simulink model "acc_plant"  (R2026b)
settings: Solver=ode3  StopTime=60  FixedStep=0.005
values from neighbouring files (symbols this model uses):
  P = min(P / (lam + pk^2 * P), P0)    [acc_mass_estimate.m]    (also in acc_plant_params.m = longitudinal_params("trailer"); acc_scenario_input.m = acc_plant_params(); build_acc_closed_loop.m = acc_plant_params(); build_acc_plant.m = acc_plant_params())
libraries: simulink x11, sl_discontinuities x2
settings Model: Creator=kikiw  LastModifiedBy=kikiw
settings DebuggingCC: AlgebraicLoopMsg=error

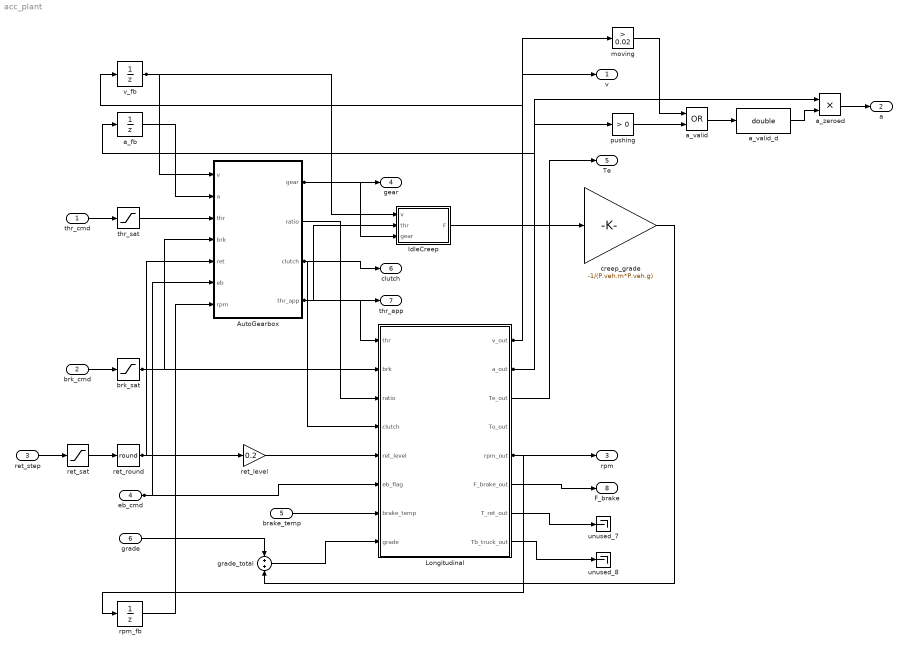
== system acc_plant ==
  thr_cmd : Inport
  brk_cmd : Inport  Port=2
  ret_step : Inport  Port=3
  eb_cmd : Inport  Port=4
  brake_temp : Inport  Port=5
  grade : Inport  Port=6
  AutoGearbox : Stateflow chart  TreatAsAtomicUnit=on
  IdleCreep : MATLAB Function  TreatAsAtomicUnit=on
  Longitudinal : Subsystem
  a_fb : UnitDelay  InitialCondition=P.init.a0  SampleTime=0.02
  a_valid : Logic  Operator=OR  AllPortsSameDT=off  OutDataTypeStr=boolean
  a_valid_d : DataTypeConversion  OutDataTypeStr=double  SaturateOnIntegerOverflow=off  RndMeth=Floor
  a_zeroed : Product
  brk_sat : Saturate  UpperLimit=1  LowerLimit=0
  creep_grade : Gain  Gain=-1/(P.veh.m*P.veh.g)
  grade_total : Sum
  moving : simulink/Logic and Bit Operations/Compare To Constant  relop=>  const=0.02  OutDataTypeStr=boolean
  pushing : simulink/Logic and Bit Operations/Compare To Constant  relop=>  const=0  OutDataTypeStr=boolean
  ret_level : Gain  Gain=0.2
  ret_round : Rounding  Operator=round
  ret_sat : Saturate  UpperLimit=5  LowerLimit=0
  rpm_fb : UnitDelay  InitialCondition=P.init.we0*30/pi  SampleTime=0.02
  thr_sat : Saturate  UpperLimit=1  LowerLimit=0
  unused_7 : Terminator
  unused_8 : Terminator
  v_fb : UnitDelay  InitialCondition=P.init.v0  SampleTime=0.02
  v : Outport
  a : Outport  Port=2
  rpm : Outport  Port=3
  gear : Outport  Port=4
  Te : Outport  Port=5
  clutch : Outport  Port=6
  thr_app : Outport  Port=7
  F_brake : Outport  Port=8
  wires:
  brk_cmd/1 -> brk_sat/1
  moving/1 -> a_valid/1
  ret_step/1 -> ret_sat/1
  AutoGearbox/2(ratio) -> Longitudinal/3(ratio)
  thr_cmd/1 -> thr_sat/1
  ret_sat/1 -> ret_round/1
  a_fb/1 -> AutoGearbox/2(a)
  v_fb/1 -> IdleCreep/1(v), AutoGearbox/1(v)
  thr_sat/1 -> AutoGearbox/3(thr)
  brk_sat/1 -> Longitudinal/2(brk), AutoGearbox/4(brk)
  ret_round/1 -> ret_level/1, AutoGearbox/5(ret)
  eb_cmd/1 -> Longitudinal/6(eb_flag), AutoGearbox/6(eb)
  Longitudinal/1(v_out) -> moving/1, v_fb/1, v/1
  grade/1 -> grade_total/1
  rpm_fb/1 -> AutoGearbox/7(rpm)
  AutoGearbox/1(gear) -> IdleCreep/3(gear), gear/1
  AutoGearbox/3(clutch) -> Longitudinal/4(clutch), clutch/1
  AutoGearbox/4(thr_app) -> Longitudinal/1(thr), IdleCreep/2(thr), thr_app/1
  a_valid_d/1 -> a_zeroed/2
  Longitudinal/8(Tb_truck_out) -> unused_8/1
  ret_level/1 -> Longitudinal/5(ret_level)
  brake_temp/1 -> Longitudinal/7(brake_temp)
  IdleCreep/1(F) -> creep_grade/1
  grade_total/1 -> Longitudinal/8(grade)
  Longitudinal/2(a_out) -> a_fb/1, a_zeroed/1, pushing/1
  Longitudinal/3(Te_out) -> Te/1
  Longitudinal/5(rpm_out) -> rpm_fb/1, rpm/1
  Longitudinal/6(F_brake_out) -> F_brake/1
  Longitudinal/7(T_ret_out) -> unused_7/1
  pushing/1 -> a_valid/2
  creep_grade/1 -> grade_total/2
  a_valid/1 -> a_valid_d/1
  a_zeroed/1 -> a/1

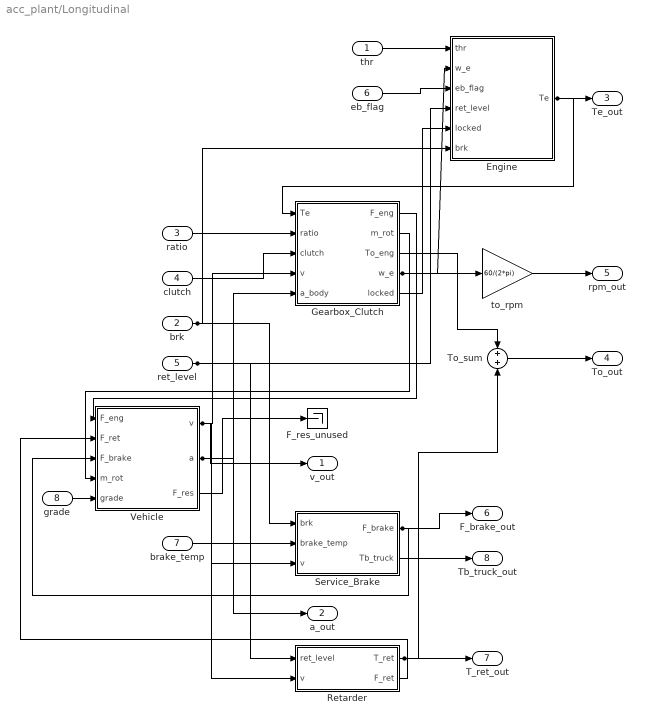
== system acc_plant/Longitudinal ==
  thr : Inport
  brk : Inport  Port=2
  ratio : Inport  Port=3
  clutch : Inport  Port=4
  ret_level : Inport  Port=5
  eb_flag : Inport  Port=6
  brake_temp : Inport  Port=7
  grade : Inport  Port=8
  Engine : Subsystem
  F_res_unused : Terminator
  Gearbox_Clutch : Subsystem
  Retarder : Subsystem
  Service_Brake : Subsystem
  To_sum : Sum
  Vehicle : Subsystem
  to_rpm : Gain  Gain=60/(2*pi)
  v_out : Outport
  a_out : Outport  Port=2
  Te_out : Outport  Port=3
  To_out : Outport  Port=4
  rpm_out : Outport  Port=5
  F_brake_out : Outport  Port=6
  T_ret_out : Outport  Port=7
  Tb_truck_out : Outport  Port=8
  wires:
  grade/1 -> Vehicle/5(grade)
  ratio/1 -> Gearbox_Clutch/2(ratio)
  clutch/1 -> Gearbox_Clutch/3(clutch)
  brk/1 -> Service_Brake/1(brk), Engine/6(brk)
  ret_level/1 -> Retarder/1(ret_level), Engine/4(ret_level)
  Vehicle/3(F_res) -> F_res_unused/1
  Vehicle/1(v) -> Gearbox_Clutch/4(v), Service_Brake/3(v), v_out/1, Retarder/2(v)
  Vehicle/2(a) -> a_out/1, Gearbox_Clutch/5(a_body)
  brake_temp/1 -> Service_Brake/2(brake_temp)
  Gearbox_Clutch/3(To_eng) -> To_sum/1
  thr/1 -> Engine/1(thr)
  eb_flag/1 -> Engine/3(eb_flag)
  Gearbox_Clutch/1(F_eng) -> Vehicle/1(F_eng)
  Gearbox_Clutch/2(m_rot) -> Vehicle/4(m_rot)
  Gearbox_Clutch/4(w_e) -> to_rpm/1, Engine/2(w_e)
  To_sum/1 -> To_out/1
  Gearbox_Clutch/5(locked) -> Engine/5(locked)
  Service_Brake/1(F_brake) -> F_brake_out/1, Vehicle/3(F_brake)
  Service_Brake/2(Tb_truck) -> Tb_truck_out/1
  Retarder/1(T_ret) -> T_ret_out/1, To_sum/2
  Retarder/2(F_ret) -> Vehicle/2(F_ret)
  Engine/1(Te) -> Te_out/1, Gearbox_Clutch/1(Te)
  to_rpm/1 -> rpm_out/1

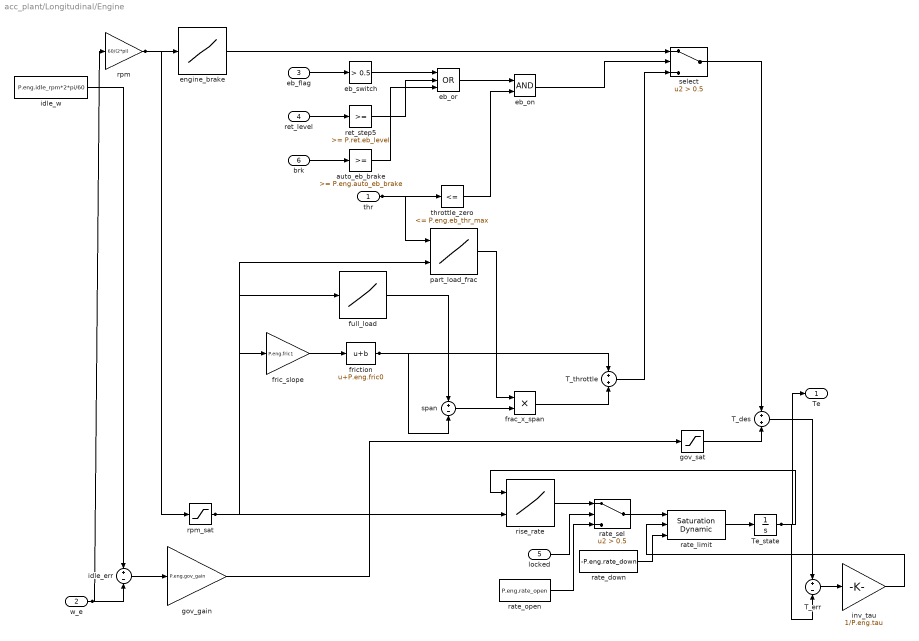
== system acc_plant/Longitudinal/Engine ==
  thr : Inport
  w_e : Inport  Port=2
  eb_flag : Inport  Port=3
  ret_level : Inport  Port=4
  locked : Inport  Port=5
  brk : Inport  Port=6
  T_des : Sum
  T_err : Sum  Inputs=+-
  T_throttle : Sum
  Te_state : Integrator  InitialCondition=P.init.Te0
  auto_eb_brake : simulink/Logic and Bit Operations/Compare To Constant  relop=>=  const=P.eng.auto_eb_brake  OutDataTypeStr=boolean
  eb_on : Logic  AllPortsSameDT=off  OutDataTypeStr=boolean
  eb_or : Logic  Operator=OR  Inputs=3  AllPortsSameDT=off  OutDataTypeStr=boolean
  eb_switch : simulink/Logic and Bit Operations/Compare To Constant  relop=>  const=0.5  OutDataTypeStr=boolean
  engine_brake : Lookup_n-D  NumberOfTableDimensions=1  BreakpointsForDimension1=P.eng.eb_rpm  Table=P.eng.eb_nm  ExtrapMethod=Clip  InternalRulePriority=Speed  RndMeth=Simplest
  frac_x_span : Product
  fric_slope : Gain  Gain=P.eng.fric1
  friction : Bias  Bias=P.eng.fric0  SaturateOnIntegerOverflow=off
  full_load : Lookup_n-D  NumberOfTableDimensions=1  BreakpointsForDimension1=P.eng.curve_rpm  Table=P.eng.T_max*P.eng.curve_frac  ExtrapMethod=Clip  InternalRulePriority=Speed  RndMeth=Simplest
  gov_gain : Gain  Gain=P.eng.gov_gain
  gov_sat : Saturate  UpperLimit=P.eng.T_max  LowerLimit=0
  idle_err : Sum  Inputs=+-
  idle_w : Constant  Value=P.eng.idle_rpm*2*pi/60
  inv_tau : Gain  Gain=1/P.eng.tau
  part_load_frac : Lookup_n-D  BreakpointsForDimension1=P.eng.thr_bp  BreakpointsForDimension2=P.eng.rpm_bp  Table=P.eng.frac_table  ExtrapMethod=Clip  InternalRulePriority=Speed  RndMeth=Simplest
      settings: InputPortMap=u0,u1
  rate_down : Constant  Value=-P.eng.rate_down
  rate_limit : sl_discontinuities/Saturation Dynamic  OutMin=[]  OutMax=[]  OutDataTypeStr=Inherit: Same as second input  OutDataType=fixdt(1, 16)  OutScaling=2^-10  DoSatur=off
      settings: LibrarySourceBlock=|
      | simulink/Discontinuities/Saturation
      | Dynamic
  rate_open : Constant  Value=P.eng.rate_open
  rate_sel : Switch  Criteria=u2 > Threshold  Threshold=0.5  SaturateOnIntegerOverflow=off  InputSameDT=off
  ret_step5 : simulink/Logic and Bit Operations/Compare To Constant  relop=>=  const=P.ret.eb_level  OutDataTypeStr=boolean
  rise_rate : Lookup_n-D  BreakpointsForDimension1=P.eng.rate_te_bp  BreakpointsForDimension2=P.eng.rate_rpm_bp  Table=P.eng.rate_up_table  ExtrapMethod=Clip  InternalRulePriority=Speed  RndMeth=Simplest
      settings: InputPortMap=u0,u1
  rpm : Gain  Gain=60/(2*pi)
  rpm_sat : Saturate  UpperLimit=P.eng.curve_rpm(end)  LowerLimit=P.eng.curve_rpm(1)
  select : Switch  Criteria=u2 > Threshold  Threshold=0.5  SaturateOnIntegerOverflow=off  InputSameDT=off
  span : Sum  Inputs=+-
  throttle_zero : simulink/Logic and Bit Operations/Compare To Constant  relop=<=  const=P.eng.eb_thr_max  OutDataTypeStr=boolean
  Te : Outport
  wires:
  inv_tau/1 -> rate_limit/2
  T_des/1 -> T_err/1
  gov_sat/1 -> T_des/2
  rate_down/1 -> rate_limit/3
  T_err/1 -> inv_tau/1
  rate_sel/1 -> rate_limit/1
  rate_open/1 -> rate_sel/3
  locked/1 -> rate_sel/2
  frac_x_span/1 -> T_throttle/2
  T_throttle/1 -> select/3
  eb_on/1 -> select/2
  rate_limit/1 -> Te_state/1
  span/1 -> frac_x_span/2
  friction/1 -> span/2, T_throttle/1
  part_load_frac/1 -> frac_x_span/1
  full_load/1 -> span/1
  thr/1 -> throttle_zero/1, part_load_frac/1
  rise_rate/1 -> rate_sel/1
  auto_eb_brake/1 -> eb_or/3
  throttle_zero/1 -> eb_on/2
  eb_switch/1 -> eb_or/1
  ret_step5/1 -> eb_or/2
  fric_slope/1 -> friction/1
  eb_or/1 -> eb_on/1
  brk/1 -> auto_eb_brake/1
  ret_level/1 -> ret_step5/1
  eb_flag/1 -> eb_switch/1
  engine_brake/1 -> select/1
  rpm/1 -> engine_brake/1, rpm_sat/1
  rpm_sat/1 -> rise_rate/2, fric_slope/1, full_load/1, part_load_frac/2
  idle_w/1 -> idle_err/1
  Te_state/1 -> T_err/2, Te/1, rise_rate/1
  idle_err/1 -> gov_gain/1
  w_e/1 -> rpm/1, idle_err/2
  select/1 -> T_des/1
  gov_gain/1 -> gov_sat/1

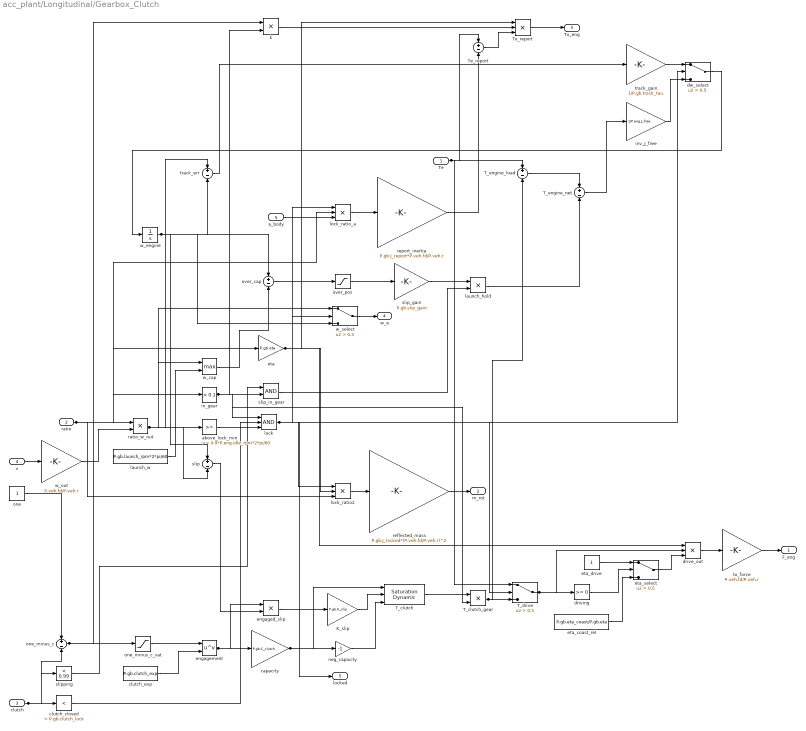
== system acc_plant/Longitudinal/Gearbox_Clutch ==
  Te : Inport
  ratio : Inport  Port=2
  clutch : Inport  Port=3
  v : Inport  Port=4
  a_body : Inport  Port=5
  K_slip : Gain  Gain=P.gb.K_slip
  T_clutch : sl_discontinuities/Saturation Dynamic  OutMin=[]  OutMax=[]  OutDataTypeStr=Inherit: Same as second input  OutDataType=fixdt(1, 16)  OutScaling=2^-10  DoSatur=off
      settings: LibrarySourceBlock=|
      | simulink/Discontinuities/Saturation
      | Dynamic
  T_clutch_gear : Product
  T_drive : Switch  Criteria=u2 > Threshold  Threshold=0.5  SaturateOnIntegerOverflow=off  InputSameDT=off
  T_engine_load : Sum  Inputs=+-
  T_engine_net : Sum  Inputs=+-
  Te_report : Sum  Inputs=+-
  To_report : Product  Inputs=3
  above_lock_min : simulink/Logic and Bit Operations/Compare To Constant  relop=>=  const=0.9*P.eng.idle_rpm*2*pi/60  OutDataTypeStr=boolean
  capacity : Gain  Gain=P.gb.C_clutch
  clutch_closed : simulink/Logic and Bit Operations/Compare To Constant  relop=<  const=P.gb.clutch_lock  OutDataTypeStr=boolean
  clutch_exp : Constant  Value=P.gb.clutch_exp
  drive_out : Product  Inputs=3
  driving : simulink/Logic and Bit Operations/Compare To Constant  relop=>=  const=0  OutDataTypeStr=boolean
  dw_select : Switch  Criteria=u2 > Threshold  Threshold=0.5  SaturateOnIntegerOverflow=off  InputSameDT=off
  engaged_slip : Product
  engagement : Math  Operator=pow
  eta : Gain  Gain=P.gb.eta
  eta_coast_rel : Constant  Value=P.gb.eta_coast/P.gb.eta
  eta_drive : Constant
  eta_select : Switch  Criteria=u2 > Threshold  Threshold=0.5  SaturateOnIntegerOverflow=off  InputSameDT=off
  in_gear : simulink/Logic and Bit Operations/Compare To Constant  relop=>  const=0.1  OutDataTypeStr=boolean
  inv_J_free : Gain  Gain=1/P.eng.J_free
  k : Product
  launch_hold : Product
  launch_w : Constant  Value=P.gb.launch_rpm*2*pi/60
  lock : Logic  Inputs=3  AllPortsSameDT=off  OutDataTypeStr=boolean
  lock_ratio2 : Product  Inputs=3
  lock_ratio_a : Product  Inputs=3
  neg_capacity : Gain  Gain=-1
  one : Constant
  one_minus_c : Sum  Inputs=+-
  one_minus_c_sat : Saturate  UpperLimit=1  LowerLimit=0
  over_cap : Sum  Inputs=+-
  over_pos : Saturate  UpperLimit=inf  LowerLimit=0
  ratio_w_out : Product
  reflected_mass : Gain  Gain=P.gb.J_locked*(P.veh.fd/P.veh.r)^2
  report_inertia : Gain  Gain=P.gb.J_report*P.veh.fd/P.veh.r
  slip : Sum  Inputs=+-
  slip_gain : Gain  Gain=P.gb.slip_gain
  slip_in_gear : Logic  AllPortsSameDT=off  OutDataTypeStr=boolean
  slipping : simulink/Logic and Bit Operations/Compare To Constant  relop=<  const=0.99  OutDataTypeStr=boolean
  to_force : Gain  Gain=P.veh.fd/P.veh.r
  track_err : Sum  Inputs=+-
  track_gain : Gain  Gain=1/P.gb.track_tau
  w_cap : MinMax  Function=max  Inputs=2
  w_engine : Integrator  InitialCondition=P.init.we0  LimitOutput=on  UpperSaturationLimit=P.eng.max_rpm*2*pi/60  LowerSaturationLimit=0
  w_out : Gain  Gain=P.veh.fd/P.veh.r
  w_select : Switch  Criteria=u2 > Threshold  Threshold=0.5  SaturateOnIntegerOverflow=off  InputSameDT=off
  F_eng : Outport
  m_rot : Outport  Port=2
  To_eng : Outport  Port=3
  w_e : Outport  Port=4
  locked : Outport  Port=5
  wires:
  drive_out/1 -> to_force/1
  dw_select/1 -> w_engine/1
  eta_select/1 -> drive_out/3
  inv_J_free/1 -> dw_select/3
  track_gain/1 -> dw_select/1
  eta_coast_rel/1 -> eta_select/3
  driving/1 -> eta_select/2
  eta_drive/1 -> eta_select/1
  T_engine_net/1 -> inv_J_free/1
  T_drive/1 -> driving/1, drive_out/2
  launch_hold/1 -> T_engine_net/2
  T_clutch/1 -> T_clutch_gear/1
  report_inertia/1 -> Te_report/2
  to_force/1 -> F_eng/1
  K_slip/1 -> T_clutch/2
  lock_ratio2/1 -> reflected_mass/1
  slip_gain/1 -> launch_hold/1
  Te_report/1 -> To_report/3
  over_pos/1 -> slip_gain/1
  lock_ratio_a/1 -> report_inertia/1
  To_report/1 -> To_eng/1
  slip_in_gear/1 -> launch_hold/2
  eta/1 -> lock_ratio2/2, To_report/1, drive_out/1
  T_clutch_gear/1 -> T_drive/3, T_engine_load/2
  over_cap/1 -> over_pos/1
  a_body/1 -> lock_ratio_a/3
  k/1 -> To_report/2
  reflected_mass/1 -> m_rot/1
  engagement/1 -> capacity/1, engaged_slip/1
  slip/1 -> engaged_slip/2
  Te/1 -> T_engine_load/1, T_drive/1, Te_report/1
  above_lock_min/1 -> lock/3
  w_cap/1 -> over_cap/2
  in_gear/1 -> k/2, slip_in_gear/2, T_clutch_gear/2, lock/1
  T_engine_load/1 -> T_engine_net/1
  track_err/1 -> track_gain/1
  lock/1 -> locked/1, T_drive/2, lock_ratio2/1, w_select/2, lock_ratio_a/1, dw_select/2
  w_select/1 -> w_e/1
  clutch_exp/1 -> engagement/2
  neg_capacity/1 -> T_clutch/3
  one_minus_c_sat/1 -> engagement/1
  launch_w/1 -> w_cap/2
  ratio_w_out/1 -> w_cap/1, above_lock_min/1, slip/2, w_select/1, track_err/1
  w_engine/1 -> slip/1, over_cap/1, w_select/3, track_err/2
  clutch_closed/1 -> lock/2
  w_out/1 -> ratio_w_out/2
  one/1 -> one_minus_c/1
  one_minus_c/1 -> one_minus_c_sat/1, k/1
  slipping/1 -> slip_in_gear/1
  v/1 -> w_out/1
  capacity/1 -> neg_capacity/1, T_clutch/1
  clutch/1 -> slipping/1, one_minus_c/2, clutch_closed/1
  engaged_slip/1 -> K_slip/1
  ratio/1 -> ratio_w_out/1, lock_ratio_a/2, lock_ratio2/3, eta/1, in_gear/1

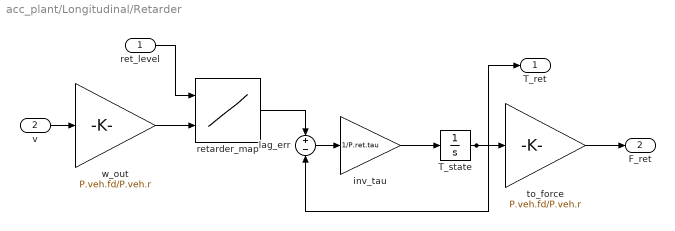
== system acc_plant/Longitudinal/Retarder ==
  ret_level : Inport
  v : Inport  Port=2
  T_state : Integrator  InitialCondition=P.init.ret0
  inv_tau : Gain  Gain=1/P.ret.tau
  lag_err : Sum  Inputs=+-
  retarder_map : Lookup_n-D  BreakpointsForDimension1=P.ret.level_bp  BreakpointsForDimension2=P.ret.w_bp  Table=P.ret.table  ExtrapMethod=Clip  InternalRulePriority=Speed  RndMeth=Simplest
      settings: InputPortMap=u0,u1
  to_force : Gain  Gain=P.veh.fd/P.veh.r
  w_out : Gain  Gain=P.veh.fd/P.veh.r
  T_ret : Outport
  F_ret : Outport  Port=2
  wires:
  ret_level/1 -> retarder_map/1
  inv_tau/1 -> T_state/1
  to_force/1 -> F_ret/1
  v/1 -> w_out/1
  w_out/1 -> retarder_map/2
  retarder_map/1 -> lag_err/1
  lag_err/1 -> inv_tau/1
  T_state/1 -> to_force/1, T_ret/1, lag_err/2

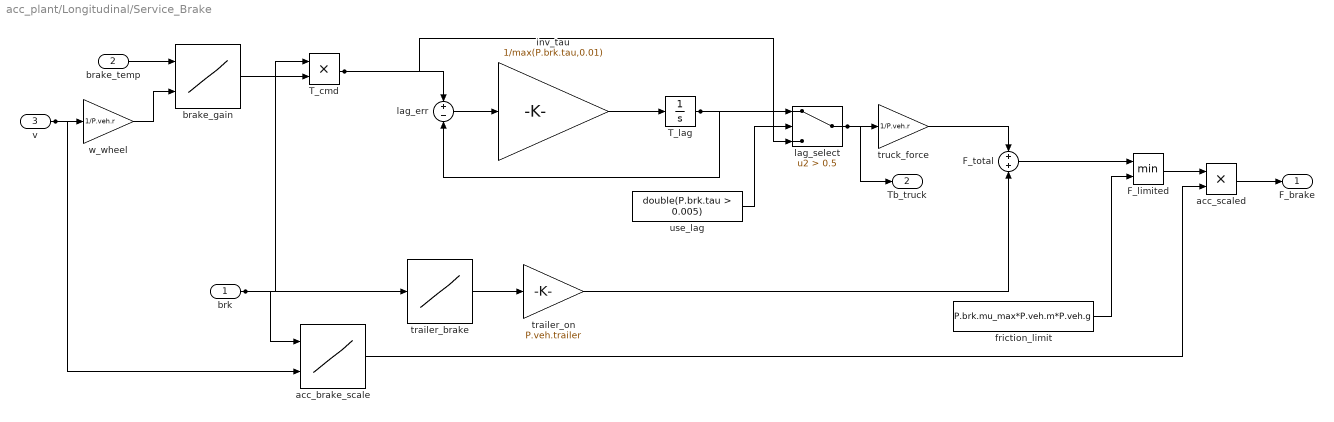
== system acc_plant/Longitudinal/Service_Brake ==
  brk : Inport
  brake_temp : Inport  Port=2
  v : Inport  Port=3
  F_limited : MinMax  Inputs=2
  F_total : Sum
  T_cmd : Product
  T_lag : Integrator
  acc_brake_scale : Lookup_n-D  BreakpointsForDimension1=P.acc.brk_b  BreakpointsForDimension2=P.acc.brk_v  Table=P.acc.brk_scale.'  ExtrapMethod=Clip  InternalRulePriority=Speed  RndMeth=Simplest
      settings: InputPortMap=u0,u1
  acc_scaled : Product
  brake_gain : Lookup_n-D  BreakpointsForDimension1=P.brk.temp_bp  BreakpointsForDimension2=P.brk.w_bp  Table=P.brk.gain_table  ExtrapMethod=Clip  InternalRulePriority=Speed  RndMeth=Simplest
      settings: InputPortMap=u0,u1
  friction_limit : Constant  Value=P.brk.mu_max*P.veh.m*P.veh.g
  inv_tau : Gain  Gain=1/max(P.brk.tau,0.01)
  lag_err : Sum  Inputs=+-
  lag_select : Switch  Criteria=u2 > Threshold  Threshold=0.5  SaturateOnIntegerOverflow=off  InputSameDT=off
  trailer_brake : Lookup_n-D  NumberOfTableDimensions=1  BreakpointsForDimension1=P.brk.trailer_bp  Table=P.brk.trailer_force  ExtrapMethod=Clip  InternalRulePriority=Speed  RndMeth=Simplest
  trailer_on : Gain  Gain=P.veh.trailer
  truck_force : Gain  Gain=1/P.veh.r
  use_lag : Constant  Value=double(P.brk.tau > 0.005)
  w_wheel : Gain  Gain=1/P.veh.r
  F_brake : Outport
  Tb_truck : Outport  Port=2
  wires:
  acc_scaled/1 -> F_brake/1
  lag_err/1 -> inv_tau/1
  use_lag/1 -> lag_select/2
  T_cmd/1 -> lag_err/1, lag_select/3
  v/1 -> acc_brake_scale/2, w_wheel/1
  brake_temp/1 -> brake_gain/1
  brake_gain/1 -> T_cmd/2
  T_lag/1 -> lag_err/2, lag_select/1
  w_wheel/1 -> brake_gain/2
  brk/1 -> T_cmd/1, trailer_brake/1, acc_brake_scale/1
  acc_brake_scale/1 -> acc_scaled/2
  F_limited/1 -> acc_scaled/1
  trailer_brake/1 -> trailer_on/1
  inv_tau/1 -> T_lag/1
  trailer_on/1 -> F_total/2
  lag_select/1 -> Tb_truck/1, truck_force/1
  truck_force/1 -> F_total/1
  F_total/1 -> F_limited/1
  friction_limit/1 -> F_limited/2

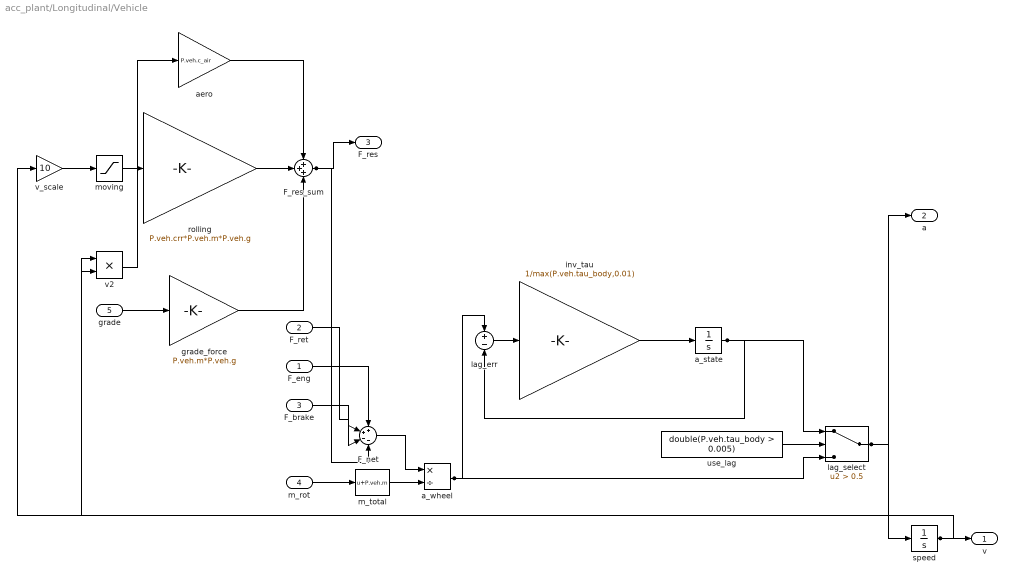
== system acc_plant/Longitudinal/Vehicle ==
  F_eng : Inport
  F_ret : Inport  Port=2
  F_brake : Inport  Port=3
  m_rot : Inport  Port=4
  grade : Inport  Port=5
  F_net : Sum  Inputs=++--
  F_res_sum : Sum  Inputs=+++
  a_state : Integrator  InitialCondition=P.init.a0
  a_wheel : Product  Inputs=*/
  aero : Gain  Gain=P.veh.c_air
  grade_force : Gain  Gain=P.veh.m*P.veh.g
  inv_tau : Gain  Gain=1/max(P.veh.tau_body,0.01)
  lag_err : Sum  Inputs=+-
  lag_select : Switch  Criteria=u2 > Threshold  Threshold=0.5  SaturateOnIntegerOverflow=off  InputSameDT=off
  m_total : Bias  Bias=P.veh.m  SaturateOnIntegerOverflow=off
  moving : Saturate  UpperLimit=1  LowerLimit=0
  rolling : Gain  Gain=P.veh.crr*P.veh.m*P.veh.g
  speed : Integrator  InitialCondition=P.init.v0  LimitOutput=on  LowerSaturationLimit=0
  use_lag : Constant  Value=double(P.veh.tau_body > 0.005)
  v2 : Product
  v_scale : Gain  Gain=10
  v : Outport
  a : Outport  Port=2
  F_res : Outport  Port=3
  wires:
  a_state/1 -> lag_select/1, lag_err/2
  lag_err/1 -> inv_tau/1
  speed/1 -> v_scale/1, v/1, v2/2, v2/1
  a_wheel/1 -> lag_err/1, lag_select/3
  F_net/1 -> a_wheel/1
  inv_tau/1 -> a_state/1
  m_rot/1 -> m_total/1
  F_brake/1 -> F_net/3
  m_total/1 -> a_wheel/2
  use_lag/1 -> lag_select/2
  F_ret/1 -> F_net/2
  lag_select/1 -> a/1, speed/1
  moving/1 -> rolling/1
  aero/1 -> F_res_sum/1
  rolling/1 -> F_res_sum/2
  v_scale/1 -> moving/1
  F_eng/1 -> F_net/1
  v2/1 -> aero/1
  grade_force/1 -> F_res_sum/3
  F_res_sum/1 -> F_res/1, F_net/4
  grade/1 -> grade_force/1

== stateflow chart acc_plant/AutoGearbox ==
  settings: updateMethod=DISCRETE  sampleTime=0.02  description=Game automatic gearbox (G33CM-R, real automatic). Fitted to acc-20261020-192243, see acc_plant_params.m. Upshift above up_rpm(thr, gear) to the highest gear that keeps >= 899/910/935 rpm (gear skipping), predictive downshift, retarder-5/engine-brake downshift to <= 2,500 rpm, neutral near standstill, launch with a clutch capacity ramp. Shift: 0.5 s open, 0.233 s close.
  state NEUTRAL
    entry: gear = 0; ratio = 0; clutch = 0; target = 0;
    during: thr_app = 0;
  state LAUNCH_ENGAGE
    entry: clutch = 1; thr_app = 0; gear = AT_launch_gear; target = gear;
  state LAUNCH_SLIP
    entry: ratio = AT_ratio(gear); tl = 0;
    during: tl = tl + AT_dt; thr_app = thr; clutch = launch_clutch();
  state DRIVE
    entry: clutch = 0;
    during: thr_app = thr; target = select_gear(gear, ret >= 4.5 || eb > 0.5);
  state LAUNCH_CLOSE
    during: thr_app = thr; clutch = max(0, clutch - AT_dt/AT_launch_t_close);
  state SHIFT_OPEN
    entry: down = double(target < gear);
    during: clutch = min(1, clutch + AT_dt/AT_t_ramp_open);
    if down > 0.5 && clutch >= 0.99, thr_app = AT_blip; else, thr_app = max(0, thr_app - AT_dt/0.1); end
  state SHIFT_CLOSE
    entry: gear = target; ratio = AT_ratio(gear);
    during: clutch = max(0, clutch - AT_dt/AT_t_close); thr_app = 0;
  state THR_RETURN
    entry: clutch = 0;
    during: thr_app = min(thr, thr_app + max(thr, 0.05)*AT_dt/AT_t_thr);
  LAUNCH_SLIP -> NEUTRAL [order 1] : [thr <= AT_creep_thr && v < 1]
  LAUNCH_ENGAGE -> NEUTRAL [order 1] : [thr <= AT_creep_thr]
  DRIVE -> NEUTRAL [order 1] : [neutral_cond(gear)]
  SHIFT_OPEN -> NEUTRAL [order 1] : [neutral_cond(gear)]
  (junction 60) -> NEUTRAL [order 2]
  NEUTRAL -> LAUNCH_ENGAGE [order 1] : [thr > AT_creep_thr && v < 2]
  DRIVE -> LAUNCH_SLIP [order 2] : [thr > AT_creep_thr && v*AT_kv*AT_ratio(gear) < AT_neutral_rpm]
  LAUNCH_ENGAGE -> LAUNCH_SLIP [order 2] : [after(AT_launch_t_engage, sec)]
  NEUTRAL -> SHIFT_CLOSE [order 2] : [v >= 2 && (thr > AT_creep_thr || (brk < 0.05 && after(0.5, sec)))]{target = engage_gear(); clutch = 1;}
  LAUNCH_CLOSE -> DRIVE : [clutch <= 0]
  LAUNCH_SLIP -> LAUNCH_CLOSE [order 2] : [thr <= AT_creep_thr || AT_ratio(gear)*v*AT_kv >= AT_launch_sync*rpm]
  THR_RETURN -> DRIVE : [after(AT_t_thr, sec)]
  (junction 60) -> DRIVE [order 1] : [AT_init_gear > 0]{gear = AT_init_gear; target = gear; ratio = AT_ratio(gear); clutch = 0;}
  (default) -> (junction 60)
  DRIVE -> SHIFT_OPEN [order 3] : [target >= 1 && target ~= gear && after(AT_dwell, sec)]
  SHIFT_OPEN -> SHIFT_CLOSE [order 2] : [after(AT_t_open, sec)]
  SHIFT_CLOSE -> THR_RETURN : [after(AT_t_close, sec)]
  data: g function_input; bm function_input; tg function_output; g function_input; y function_output; c function_output; g function_output; v input; a input; thr input; brk input; ret input; eb input; rpm input; gear output =0; ratio output =0; clutch output =0; thr_app output =0; target local =0; down local =0; tl local =0; AT_ratio parameter; AT_kv parameter; AT_dt parameter; AT_top_gear parameter; AT_min_gear parameter; AT_up_thr parameter; AT_up_rpm parameter; AT_up_slope parameter; AT_up_min parameter; AT_dn0 parameter; AT_dn0_thr parameter; AT_dn_slope parameter; AT_dn_slope_thr parameter; AT_t_pred parameter; AT_dn_target parameter; AT_eb_trig parameter; AT_eb_max parameter; AT_neutral_rpm parameter; AT_neutral_brk parameter; AT_neutral_brk_rpm parameter; AT_t_open parameter; AT_t_ramp_open parameter; AT_t_close parameter; AT_t_thr parameter; AT_blip parameter; AT_dwell parameter; AT_launch_gear parameter; AT_launch_thr parameter; AT_launch_t_engage parameter; AT_launch_t_close parameter; AT_launch_sync parameter; AT_launch_cap_max parameter; AT_launch_cap_t parameter; AT_C_clutch parameter; AT_clutch_exp parameter; AT_creep_thr parameter; AT_init_gear parameter
  function tg = select_gear(g, bm):
    | function tg = select_gear(g, bm)
    | % Target SDK gear from the chart inputs v, a, thr. bm: retarder step 5 or engine brake.
    | tg = g;
    | if g < 1, return; end
    | r = AT_ratio;
    | vp = max(0, v + min(a, 0)*AT_t_pred);
    | rpm_now = v*AT_kv*r(g);
    | rpm_pred = vp*AT_kv*r(g);
    | if bm
    |     if rpm_now < AT_eb_trig
    |         for k = AT_min_gear:(g - 1)
    |             if v*AT_kv*r(k) <= AT_eb_max
    |                 tg = k; return;
    |             end
    |         end
    |     end
    |     return;
    | end
    | th = min(max(thr, 0), 1);
    | dn = AT_dn0 + th^3*AT_dn0_thr - (AT_dn_slope + th^3*AT_dn_slope_thr)*(12 - g);
    | if rpm_pred < dn && g > AT_min_gear
    |     tg = AT_min_gear;
    |     for k = (g - 1):-1:AT_min_gear
    |         if vp*AT_kv*r(k) >= AT_dn_target
    |             tg = k; return;
    |         end
    |     end
    |     return;
    | end
    | up = interp1(AT_up_thr, AT_up_rpm, th) - interp1(AT_up_thr, AT_up_slope, th)*(g - 4);
    | if rpm_now > up && a > -1.0 && g < AT_top_gear
    |     % the target follows from the threshold speed, not from the sampled one (the game's
    |     % choice is within a few rpm of the limits, see acc_plant_params.m)
    |     ru = up;
    |     if rpm_now > up + 30, ru = rpm_now; end
    |     tg = g + 1;
    |     for k = AT_top_gear:-1:(g + 1)
    |         lim = AT_up_min(min(k, numel(AT_up_min)));
    |         if ru*r(k)/r(g) >= lim
    |             tg = k; return;
    |         end
    |     end
    | end
  function y = neutral_cond(g):
    | function y = neutral_cond(g)
    | % The clutch opens (gear 0) near standstill or early under strong braking.
    | y = false;
    | if g < 1 || thr > 0.05, return; end
    | rpm_now = v*AT_kv*AT_ratio(g);
    | vp = max(0, v + min(a, 0)*AT_t_pred);
    | if rpm_now < AT_neutral_rpm
    |     y = true;
    | elseif brk >= AT_neutral_brk && vp*AT_kv*AT_ratio(g) < AT_neutral_brk_rpm
    |     y = true;
    | end
  function c = launch_clutch:
    | function c = launch_clutch()
    | % Clutch command while slipping: capacity ramps to cap_max(thr) in cap_t(thr) seconds (fit).
    | th = min(max(thr, 0), 1);
    | cap = interp1(AT_launch_thr, AT_launch_cap_max, th)*min(1, tl/interp1(AT_launch_thr, AT_launch_cap_t, th));
    | e = min(1, cap/AT_C_clutch);
    | c = 1 - e^(1/AT_clutch_exp);
  function g = engage_gear:
    | function g = engage_gear()
    | % Gear to engage when rolling in neutral: the highest one with >= 1,100 rpm.
    | g = AT_min_gear;
    | for k = AT_top_gear:-1:AT_min_gear
    |     if v*AT_kv*AT_ratio(k) >= 1100
    |         g = k; return;
    |     end
    | end

== matlab function acc_plant/IdleCreep ==
  data: v input; F output; thr input; gear input; P parameter
function F = IdleCreep(v, thr, gear, P)
% creep force (N) of the automatic: after rolling in gear (v > creep_on_v) with the throttle
% closed, the clutch keeps slipping at idle and pushes until the truck stands still
% (v < creep_off_v: the clutch opens, docs/31 정차 유지: no creep from standstill)
persistent rolling
if isempty(rolling), rolling = false; end
if gear >= 1 && v > P.acc.creep_on_v, rolling = true; end
if v < P.acc.creep_off_v, rolling = false; end
F = 0;
if rolling && thr < 0.02
    F = P.acc.creep_force * min(max((P.acc.creep_v_zero - v) / (P.acc.creep_v_zero - P.acc.creep_v_full), 0), 1);
end
